simulink model "Maneuver"  (R2023b)
settings: Solver=ode4  StartTime=0.0  StopTime=30  FixedStep=dt  RelTol=1e-3
InitFcn:
  | SimulationInitialization
StopFcn:
  | SimulationEnd
values from neighbouring files (symbols this model uses):
  C = GeneticOpt.C    [SimulationCostFunction.m]
  c = Sw/b    (= 0.841696750903)    [SimulationControlConfig16P.m]    (also in SimulationControlConfig16P_LEGACY.m; SimulationControlConfigTAILLESS.m = 0.354008438819; SimulationControlConfigUTAIL.m = 0.354008438819)
  CL_Limit = CL_Max    (= 0.54)    [SimulationControlConfig16P.m]    (also in SimulationControlConfig16P_LEGACY.m; SimulationControlConfigTAILLESS.m; SimulationControlConfigUTAIL.m = 0.53)
  CL_Max_Nom = 0.465    [SimulationControlConfig16P.m]    (also in SimulationControlConfig16P_LEGACY.m; SimulationControlConfigTAILLESS.m = 0.39; SimulationControlConfigUTAIL.m)
  CL_Min = 0    [SimulationControlConfig16P.m]    (also in SimulationControlConfig16P_LEGACY.m; SimulationControlConfigTAILLESS.m; SimulationControlConfigUTAIL.m)
  dCl_per_dFlap = 0.005581818    [SimulationControlConfig16P.m]    (also in SimulationControlConfig16P_LEGACY.m = 0; SimulationControlConfigTAILLESS.m = 0; SimulationControlConfigUTAIL.m = 0)
  dt = DLLSim.dt    [SimulationTimeStep.m]    (also in SimulationTrim.m = 0.02)
  ElevatorDeflectionRate = 15    [SimulationControlConfig16P.m]    (also in SimulationControlConfig16P_LEGACY.m = 12; SimulationControlConfigTAILLESS.m = 10; SimulationControlConfigUTAIL.m = 12)
  ElevatorMax = 25    [SimulationControlConfig16P.m]    (also in SimulationControlConfig16P_LEGACY.m; SimulationControlConfigTAILLESS.m; SimulationControlConfigUTAIL.m)
  ElevatorPower = -0.002209    [SimulationControlConfig16P.m]    (also in SimulationControlConfig16P_LEGACY.m; SimulationControlConfigTAILLESS.m = -0.002956; SimulationControlConfigUTAIL.m = -0.00205983)
  ElevatorTrim = -3.5    [SimulationControlConfig16P.m]    (also in SimulationControlConfig16P_LEGACY.m; SimulationControlConfigTAILLESS.m = -6; SimulationControlConfigUTAIL.m = -8)
  Fp_Elevator = 0.55*2*pi*PitchRateLpfCutoff*dt    [SimulationControlConfig16P.m]    (also in SimulationControlConfig16P_LEGACY.m; SimulationControlConfigTAILLESS.m; SimulationControlConfigUTAIL.m)
  Fp_Pitch_2 = 0.55*2*pi*PitchBandwidth*dt    [SimulationControlConfig16P.m]    (also in SimulationControlConfig16P_LEGACY.m; SimulationControlConfigTAILLESS.m; SimulationControlConfigUTAIL.m)
  LaunchRollingElevator = -1.5    [SimulationControlConfig16P.m]    (also in SimulationControlConfig16P_LEGACY.m; SimulationControlConfigTAILLESS.m = 1; SimulationControlConfigUTAIL.m = 1)
  LiftSlope = 0.064285    [SimulationControlConfig16P.m]    (also in SimulationControlConfig16P_LEGACY.m; SimulationControlConfigTAILLESS.m = 0.058631; SimulationControlConfigUTAIL.m)
  LPFclestInit = 0    [SimulationControlPre.m]
  LPFvRate2PitchInit = 0.1    [SimulationControlPre.m]
  m = 13.1784    [InertiaEstimatorBWB.m]    (also in SimulationControlConfig16P.m = MassBWB; SimulationControlConfig16P_LEGACY.m = MassBWB; SimulationControlConfigTAILLESS.m = Weight / 2.2; SimulationControlConfigUTAIL.m = Weight / 2.2)
  nMax_User = 2.6    [SimulationControlConfig16P.m]    (also in SimulationControlConfig16P_LEGACY.m; SimulationControlConfigTAILLESS.m = 2.5; SimulationControlConfigUTAIL.m = 2.5)
  nMin_User = -1.3    [SimulationControlConfig16P.m]    (also in SimulationControlConfig16P_LEGACY.m; SimulationControlConfigTAILLESS.m = -1; SimulationControlConfigUTAIL.m = -1)
  Pitch2ElevatorIntegratorInit = -4    [SimulationControlPre.m]
  PitchDamping = -1.2608    [SimulationControlConfig16P.m]    (also in SimulationControlConfig16P_LEGACY.m; SimulationControlConfigTAILLESS.m = -0.6814; SimulationControlConfigUTAIL.m)
  PitchDampingTrust = 0.3    [SimulationControlConfig16P.m]    (also in SimulationControlConfig16P_LEGACY.m = 0.2; SimulationControlConfigTAILLESS.m = 0; SimulationControlConfigUTAIL.m = 0)
  PitchMaxAccel = 1.0    (= 1)    [SimulationControlConfig16P.m]    (also in SimulationControlConfig16P_LEGACY.m = 1.2; SimulationControlConfigTAILLESS.m; SimulationControlConfigUTAIL.m = 1.1)
  PitchRateLpfCutoff = 3    [SimulationControlConfig16P.m]    (also in SimulationControlConfig16P_LEGACY.m; SimulationControlConfigTAILLESS.m; SimulationControlConfigUTAIL.m = 5)
  PitchRateMax_User = PitchRateMax_User/180*pi    (= 0.523598775598)    [SimulationControlConfig16P.m]    (also in SimulationControlConfig16P_LEGACY.m; SimulationControlConfigTAILLESS.m; SimulationControlConfigUTAIL.m)
  PitchStiffness = -0.0041    [SimulationControlConfig16P.m]    (also in SimulationControlConfig16P_LEGACY.m; SimulationControlConfigTAILLESS.m = -0.00225; SimulationControlConfigUTAIL.m = -0.00194915)
  Q = GeneticOpt.Q    [SimulationCostFunction.m]
  R = GeneticOpt.R    [SimulationCostFunction.m]
  RateLimitPitchRateAccel = 0    [SimulationControlPre.m]
  RollingElevator = 5    [SimulationControlConfig16P.m]    (also in SimulationControlConfig16P_LEGACY.m; SimulationControlConfigTAILLESS.m = 6.5; SimulationControlConfigUTAIL.m = 7)
  RotationElevator = -6.5    [SimulationControlConfig16P.m]    (also in SimulationControlConfig16P_LEGACY.m; SimulationControlConfigTAILLESS.m = -4.25; SimulationControlConfigUTAIL.m = -5.7)
  RotationRate = (RotationElevator - LaunchRollingElevator)/RotationTime    (= -1)    [SimulationControlConfig16P.m]    (also in SimulationControlConfig16P_LEGACY.m; SimulationControlConfigTAILLESS.m = -1.5; SimulationControlConfigUTAIL.m = -1.86111111111)
  Sw = 4.663    [SimulationControlConfig16P.m]    (also in SimulationControlConfig16P_LEGACY.m; SimulationControlConfigTAILLESS.m = 0.839; SimulationControlConfigUTAIL.m = 0.839)
  taxiTrackOffset = testPlans(testIndx).rolloutTrackOffset    [SimulationControlConfig16P.m]    (also in SimulationControlConfig16P_LEGACY.m; SimulationControlConfigTAILLESS.m; SimulationControlConfigUTAIL.m)
  YInertia = 134.120    (= 134.12)    [SimulationControlConfig16P.m]    (also in SimulationControlConfig16P_LEGACY.m; SimulationControlConfigTAILLESS.m = IYY / 3417.17; SimulationControlConfigUTAIL.m = IYY / 3417.17)
undefined symbols (not defined in the file or in its folder): DiscIntNeverNeededParam, gain_resolution, K_TS, KI_Pitch, KP_Pitch, PB, pilotTime, stepTime
libraries: simulink x22, Lib_Piccolo x18, simulink_extras x1
(part 1 of 2)
settings Model: Creator=JSheng  LastModifiedBy=JCdFFigueira
settings SolverCC: AlgebraicLoopSolver=TrustRegion
settings DataIOCC: SaveFormat=Array  SignalLogging=off  DSMLogging=off  SaveTime=off  ReturnWorkspaceOutputs=off  OutputSaveName=COST
settings DebuggingCC: UnconnectedInputMsg=warning  UnconnectedOutputMsg=warning  UnconnectedLineMsg=warning  ArithmeticOperatorsInVariantConditions=warning
settings ModelReferenceCC: EnableRefExpFcnMdlSchedulingChecks=on
settings SFSimCC: CustomCodeUndefinedFunction=UseInterfaceOnly

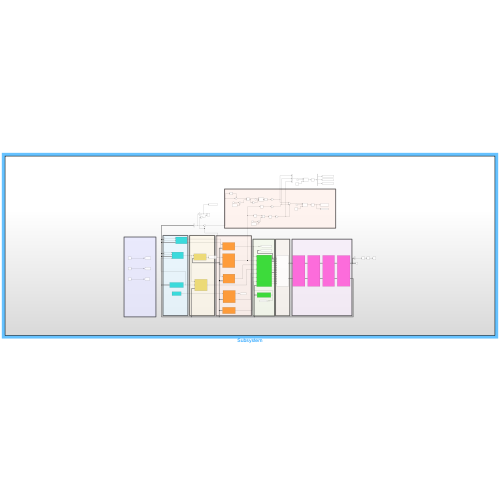
[thumbnail: Simulink's stored preview of the top-level diagram]
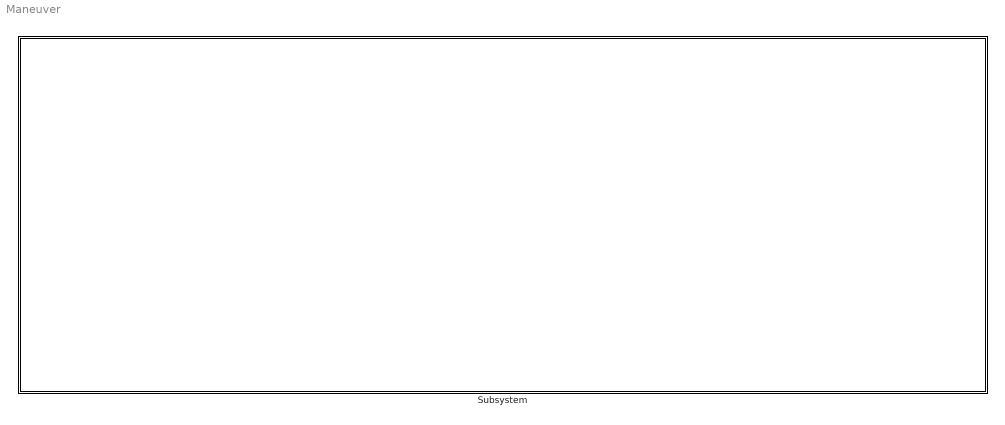
== system Maneuver ==
  Subsystem : Subsystem

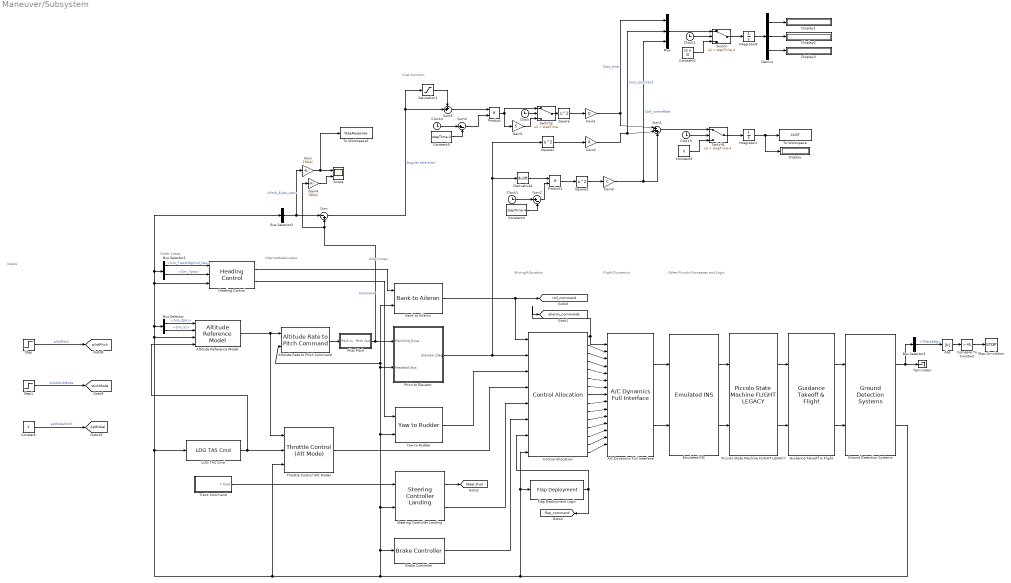
== system Maneuver/Subsystem ==
  note: Outer Loops
  note: Intermediate Loops
  note: Inner Loops
  note: Flight Dynamics
  note: Other Piccolo Processes and Logic
  note: Mixing/Allocation
  note: Inputs
  note: Cost function
  A/C Dynamics Full Interface : Lib_Piccolo/A//C Dynamics Full Interface  SystemSampleTime=-1  VariantActivationTime=update diagram  AllowFlexibleInterface=on  Latency=0  AutoFrameSizeCalculation=off
  Abs : Abs  SaturateOnIntegerOverflow=off
  Altitude Rate to Pitch Command : Lib_Piccolo/Altitude Rate to Pitch Command  SystemSampleTime=-1  VariantActivationTime=update diagram  AllowFlexibleInterface=on  Latency=0  AutoFrameSizeCalculation=off
  Altitude Reference Model : Lib_Piccolo/Altitude Reference Model  SystemSampleTime=-1  VariantActivationTime=update diagram  AllowFlexibleInterface=on  Latency=0  AutoFrameSizeCalculation=off
  Bank to Aileron : Lib_Piccolo/Bank to Aileron  SystemSampleTime=-1  VariantActivationTime=update diagram  AllowFlexibleInterface=on  Latency=0  AutoFrameSizeCalculation=off
  Brake Controller : Lib_Piccolo/Brake Controller  SystemSampleTime=-1  VariantActivationTime=update diagram  AllowFlexibleInterface=on  Latency=0  AutoFrameSizeCalculation=off
  Bus Selector : BusSelector  OutputSignals=Sim_Zpos,Sim_Vz
  Bus Selector1 : BusSelector  OutputSignals=Sim_TrackHdgCmd_Deg,Sim_Ypos
  Bus Selector2 : BusSelector  OutputSignals=Pitch_Euler_rad
  Bus Selector3 : BusSelector  OutputSignals=ThetaDeg
  Clock{,1..4} (5 alike) : Clock
  Compare To Constant : simulink/Logic and Bit Operations/Compare To Constant  relop=>  const=45  OutDataTypeStr=boolean
  Constant : Constant
  Constant2 : Constant  Value=[0 0 0]
  Constant3 : Constant  Value=0
  Constant4 : Constant  Value=stepTime-4
  Constant5 : Constant  Value=stepTime-4
  Control Allocation : Lib_Piccolo/Control Allocation  SystemSampleTime=-1  VariantActivationTime=update diagram  AllowFlexibleInterface=on  Latency=0  AutoFrameSizeCalculation=off
  Demux : Demux  Outputs=3
  Derivative1 : Derivative
  Display{,1..3} (4 alike) : Display
  Emulated INS : Lib_Piccolo/Emulated INS  SystemSampleTime=-1  VariantActivationTime=update diagram  AllowFlexibleInterface=on  Latency=0  AutoFrameSizeCalculation=off
  Flap Deployment Logic : Lib_Piccolo/Flap Deployment  SystemSampleTime=-1  VariantActivationTime=update diagram  AllowFlexibleInterface=on  Latency=0  AutoFrameSizeCalculation=off
  Gain : Gain  Gain=180/pi
  Gain1 : Gain  Gain=Q
  Gain2 : Gain  Gain=R
  Gain3 : Gain  Gain=C
  Gain4 : Gain  Gain=180/pi
  Gain5 : Gain  Gain=5
  Ground Detection Systems : Lib_Piccolo/Ground Detection Systems  SystemSampleTime=-1  VariantActivationTime=update diagram  AllowFlexibleInterface=on  Latency=0  AutoFrameSizeCalculation=off
  Guidance Takeoff & Flight : Lib_Piccolo/Guidance Takeoff & Flight  SystemSampleTime=-1  VariantActivationTime=update diagram  AllowFlexibleInterface=on  Latency=0  AutoFrameSizeCalculation=off
  Heading Control : Lib_Piccolo/Heading Control  SystemSampleTime=-1  VariantActivationTime=update diagram  AllowFlexibleInterface=on  Latency=0  AutoFrameSizeCalculation=off
  Integrator1 : Integrator
  Integrator6 : Integrator
  LDG TAS Cmd : Lib_Piccolo/LDG TAS Cmd  SystemSampleTime=-1  VariantActivationTime=update diagram  AllowFlexibleInterface=on  Latency=0  AutoFrameSizeCalculation=off
  Mux : Mux  Inputs=3
  Piccolo State Machine FLIGHT LEGACY : Lib_Piccolo/Piccolo State Machine FLIGHT LEGACY  SystemSampleTime=-1  VariantActivationTime=update diagram  AllowFlexibleInterface=on  Latency=0  AutoFrameSizeCalculation=off
  Pilot Pitch : Subsystem
  Pitch to Elevator : Subsystem  AncestorBlock=Lib_Piccolo/Pitch to Elevator
  Product : Product
  Product1 : Product
  Saturation1 : Saturate  UpperLimit=0  LowerLimit=-inf
  Scope : Scope  NumInputPorts=2
  Square : Math  Operator=square
  Square1 : Math  Operator=square
  Square2 : Math  Operator=square
  Steering Controller Landing : Lib_Piccolo/Steering Controller Landing  SystemSampleTime=-1  VariantActivationTime=update diagram  AllowFlexibleInterface=on  Latency=0  AutoFrameSizeCalculation=off
  Step : Step  Time=stepTime  Before=4.97  After=6.97  SampleTime=dt
  Step1 : Step  Time=pilotTime  SampleTime=dt
  Stop Simulation : Stop
  Sum : Sum  Inputs=|-+
  Sum1 : Sum  Inputs=|+++
  Sum2 : Sum  Inputs=|+-
  Sum3 : Sum  Inputs=++|
  Sum4 : Sum  Inputs=|+-
  Switch : Switch  Criteria=u2 > Threshold  Threshold=stepTime-4  SaturateOnIntegerOverflow=off  InputSameDT=off
  Switch1 : Switch  Criteria=u2 > Threshold  Threshold=stepTime-4  SaturateOnIntegerOverflow=off  InputSameDT=off
  Switch2 : Switch  Criteria=u2 > Threshold  Threshold=stepTime  SaturateOnIntegerOverflow=off  InputSameDT=off
  Terminator : Terminator
  Throttle Control (Alt Mode) : Lib_Piccolo/Throttle Control (Alt Mode)  SystemSampleTime=-1  VariantActivationTime=update diagram  AllowFlexibleInterface=on  Latency=0  AutoFrameSizeCalculation=off
  To Workspace : ToWorkspace  VariableName=COST  SaveFormat=Timeseries  SampleTime=-1
  To Workspace1 : ToWorkspace  VariableName=StepResponse  SaveFormat=Timeseries  SampleTime=-1
  Track Command : Subsystem
  Yaw to Rudder : Lib_Piccolo/Yaw to Rudder  SystemSampleTime=-1  VariantActivationTime=update diagram  AllowFlexibleInterface=on  Latency=0  AutoFrameSizeCalculation=off
  tag scope: ApGlobal=global, Steer_Rud=global, aileron_commands=global, flap_command=global, pilotPitch=global, roll_command=global, stickMode=global
  wires:
  Bus Selector/2 -> Altitude Reference Model/2  "<Sim_Vz>"
  Control Allocation/6 -> A/C Dynamics Full Interface/6
  Control Allocation/9 -> A/C Dynamics Full Interface/9
  Control Allocation/7 -> A/C Dynamics Full Interface/7
  Control Allocation/8 -> A/C Dynamics Full Interface/8
  Ground Detection Systems/2 -> LDG TAS Cmd/1, Bus Selector/1, Heading Control/3, Bus Selector2/1, Bus Selector1/1, Altitude Reference Model/3, Throttle Control (Alt Mode)/3, Bank to Aileron/2, Altitude Rate to Pitch Command/2, Pitch to Elevator/2(Feedback Bus), Yaw to Rudder/2, Steering Controller Landing/2, Brake Controller/1, Flap Deployment Logic/1, Control Allocation/8
  Control Allocation/3 -> A/C Dynamics Full Interface/3
  Control Allocation/11 -> A/C Dynamics Full Interface/11
  A/C Dynamics Full Interface/2 -> Emulated INS/2
  Bus Selector/1 -> Altitude Reference Model/1  "<Sim_Zpos>"
  Control Allocation/4 -> A/C Dynamics Full Interface/4
  Flap Deployment Logic/1 -> [flap_command], Control Allocation/7
  Control Allocation/13 -> A/C Dynamics Full Interface/13
  Heading Control/2 -> Yaw to Rudder/1
  Control Allocation/5 -> A/C Dynamics Full Interface/5
  A/C Dynamics Full Interface/1 -> Emulated INS/1
  Control Allocation/14 -> A/C Dynamics Full Interface/14
  Piccolo State Machine FLIGHT LEGACY/2 -> Guidance Takeoff & Flight/2
  Bus Selector1/1 -> Heading Control/1  "<Sim_TrackHdgCmd_Deg>"
  Steering Controller Landing/1 -> [Steer_Rud]
  LDG TAS Cmd/1 -> Throttle Control (Alt Mode)/2, Altitude Reference Model/4
  Brake Controller/1 -> Control Allocation/6
  Altitude Rate to Pitch Command/1 -> Pilot Pitch/1(Pitch In)
  Track Command/1(Y Cmd) -> Steering Controller Landing/1
  Emulated INS/1 -> Piccolo State Machine FLIGHT LEGACY/1
  Control Allocation/2 -> A/C Dynamics Full Interface/2
  Guidance Takeoff & Flight/1 -> Ground Detection Systems/1
  Emulated INS/2 -> Piccolo State Machine FLIGHT LEGACY/2
  Piccolo State Machine FLIGHT LEGACY/1 -> Guidance Takeoff & Flight/1
  Control Allocation/12 -> A/C Dynamics Full Interface/12
  Control Allocation/10 -> A/C Dynamics Full Interface/10
  Guidance Takeoff & Flight/2 -> Ground Detection Systems/2
  Bus Selector1/2 -> Heading Control/2  "<Sim_Ypos>"
  Control Allocation/15 -> A/C Dynamics Full Interface/15
  Steering Controller Landing/2 -> Control Allocation/5
  Ground Detection Systems/1 -> Bus Selector3/1, Terminator/1
  Control Allocation/1 -> [aileron_commands], A/C Dynamics Full Interface/1
  Bank to Aileron/1 -> Control Allocation/1, [roll_command]
  Pitch to Elevator/1(Elevator_Deg) -> Square1/1, Derivative1/1, Control Allocation/2
  Yaw to Rudder/1 -> Control Allocation/3
  Throttle Control (Alt Mode)/1 -> Control Allocation/4
  Heading Control/1 -> Bank to Aileron/1
  Altitude Reference Model/1 -> Altitude Rate to Pitch Command/1, Throttle Control (Alt Mode)/1
  Constant/1 -> [ApGlobal]  "apGlobalCmd"
  Step/1 -> [pilotPitch]  "pilotPitch"
  Step1/1 -> [stickMode]  "pilotStickMode"
  Pilot Pitch/1(Pitch Out) -> Pitch to Elevator/1(PitchCmd_Euler), Gain4/1, Sum/2  "Command"
  Saturation1/1 -> Sum3/1
  Square2/1 -> Gain3/1
  Square1/1 -> Gain2/1
  Gain1/1 -> Mux/1, Sum1/1  "Cost_error"
  Sum/1 -> Sum3/2, Saturation1/1  "Angular rate error"
  Product1/1 -> Square2/1
  Gain3/1 -> Mux/3, Sum1/3  "Cost_commRate"
  Square/1 -> Gain1/1
  Clock1/1 -> Sum2/1
  Product/1 -> Gain5/1, Switch2/1
  Derivative1/1 -> Product1/1
  Gain2/1 -> Mux/2, Sum1/2  "Cost_command"
  Bus Selector2/1 -> Gain/1, Sum/1  "<Pitch_Euler_rad>"
  Clock2/1 -> Switch/2
  Constant2/1 -> Switch/3
  Mux/1 -> Switch/1
  Integrator6/1 -> Demux/1
  Demux/1 -> Display1/1
  Demux/2 -> Display2/1
  Demux/3 -> Display3/1
  Constant3/1 -> Switch1/3
  Clock3/1 -> Switch1/2
  Sum1/1 -> Switch1/1
  Integrator1/1 -> Display/1, To Workspace/1
  Sum2/1 -> Product1/2
  Constant4/1 -> Sum2/2
  Clock4/1 -> Sum4/1
  Sum4/1 -> Product/2
  Constant5/1 -> Sum4/2
  Gain/1 -> To Workspace1/1, Scope/1
  Gain4/1 -> Scope/2
  Bus Selector3/1 -> Abs/1  "<ThetaDeg>"
  Compare To Constant/1 -> Stop Simulation/1
  Abs/1 -> Compare To Constant/1
  Sum3/1 -> Product/1
  Switch/1 -> Integrator6/1
  Switch1/1 -> Integrator1/1
  Clock/1 -> Switch2/2
  Switch2/1 -> Square/1
  Gain5/1 -> Switch2/3

== system Maneuver/Subsystem/Pilot Pitch ==
  Pitch In : Inport
  Degrees to Radians1 : simulink_extras/Transformations/Degrees to Radians
  Switch3 : Switch  Criteria=u2 > Threshold  SaturateOnIntegerOverflow=off  InputSameDT=off
  Pitch Out : Outport  VectorParamsAs1DForOutWhenUnconnected=off
  wires:
  [stickMode] -> Switch3/2
  Degrees to Radians1/1 -> Switch3/1
  Pitch In/1 -> Switch3/3
  [pilotPitch] -> Degrees to Radians1/1
  Switch3/1 -> Pitch Out/1

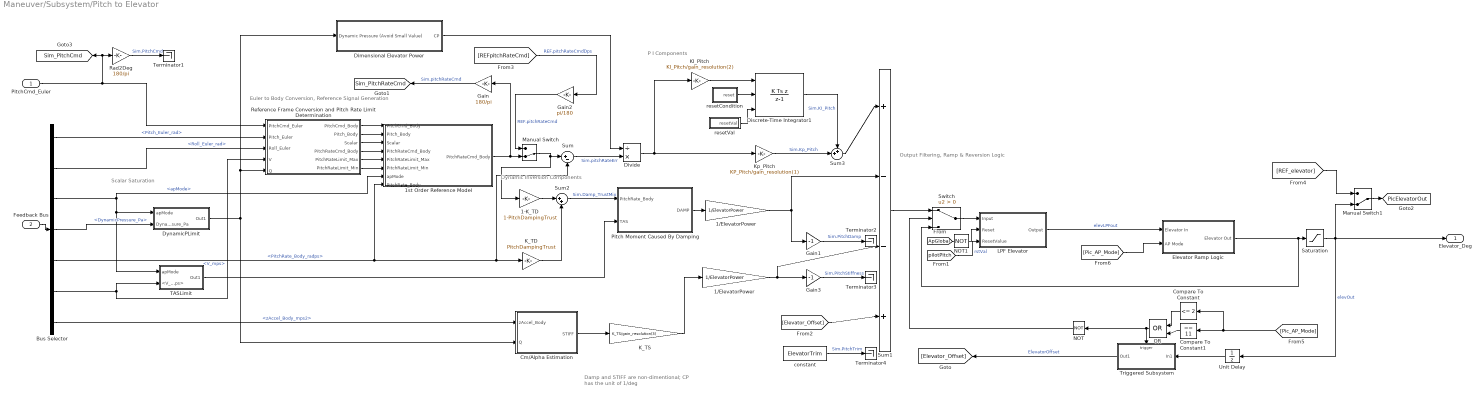
== system Maneuver/Subsystem/Pitch to Elevator ==
  note: Damp and STIFF are non-dimentional;
      | CP has the unit of 1/deg
  note: P I Components
  note: Dynamic Inversion Components
  note: Output Filtering, Ramp & Reversion Logic
  note: Scalar Saturation
  note: Euler to Body Conversion, Reference Signal Generation
  PitchCmd_Euler : Inport
  Feedback Bus : Inport  Port=2
  1-K_TD : Gain  Gain=1-PitchDampingTrust
  1/ElevatorPower : Gain  Gain=1/ElevatorPower
  "1/ElevatorPower  " : Gain  Gain=1/ElevatorPower
  1st Order Reference Model : Subsystem
  Bus Selector : BusSelector  OutputSignals=Pitch_Euler_rad,Roll_Euler_rad,apMode,DynamicPressure_Pa,PitchRate_Body_radps,V_mps,zAccel_Body_mps2
  Cm/Alpha Estimation : Subsystem
  Compare To Constant : simulink/Logic and Bit Operations/Compare To Constant  relop=<=  const=2  OutDataTypeStr=boolean
  Compare To Constant1 : simulink/Logic and Bit Operations/Compare To Constant  relop===  const=11  OutDataTypeStr=uint8
  Dimensional Elevator Power : Subsystem
  Discrete-Time Integrator1 : DiscreteIntegrator  IntegratorMethod=Integration: Backward Euler  ExternalReset=level  InitialConditionSource=external  SampleTime=-1  LimitOutput=on  UpperSaturationLimit=ElevatorMax  LowerSaturationLimit=-ElevatorMax  ICPrevOutput=DiscIntNeverNeededParam  ICPrevScaledInput=DiscIntNeverNeededParam
  Divide : Product  Inputs=/*
  DynamicPLimit : Subsystem
  Elevator Ramp Logic : Subsystem
  Gain : Gain  Gain=180/pi
  Gain1 : Gain  Gain=-1
  Gain2 : Gain  Gain=pi/180
  Gain3 : Gain  Gain=-1
  KI_Pitch : Gain  Gain=KI_Pitch/gain_resolution(2)
  K_TD : Gain  Gain=PitchDampingTrust
  K_TS : Gain  Gain=K_TS/gain_resolution(3)
  Kp_Pitch : Gain  Gain=KP_Pitch/gain_resolution(1)
  LPF Elevator : Subsystem
  Manual Switch : ManualSwitch  CurrentSetting=0
  Manual Switch1 : ManualSwitch  CurrentSetting=0
  NOT : Logic  Operator=NOT  IconShape=distinctive  AllPortsSameDT=off  OutDataTypeStr=boolean
  NOT1 : Logic  Operator=NOT  IconShape=distinctive  AllPortsSameDT=off  OutDataTypeStr=boolean
  OR : Logic  Operator=OR  IconShape=distinctive  AllPortsSameDT=off  OutDataTypeStr=boolean
  Pitch Moment Caused By Damping : Subsystem
  Rad2Deg : Gain  Gain=180/pi
  Reference Frame Conversion and Pitch Rate Limit Determination : Subsystem
  Saturation : Saturate  UpperLimit=ElevatorMax  LowerLimit=-ElevatorMax
  Sum : Sum  Inputs=|+-
  Sum1 : Sum  Inputs=|+--+
  Sum2 : Sum  Inputs=|++
  Sum3 : Sum  Inputs=++|
  Switch : Switch  Criteria=u2 > Threshold  SaturateOnIntegerOverflow=off  InputSameDT=off
  TASLimit : Subsystem
  Terminator{1..4} (4 alike) : Terminator
  Triggered Subsystem : Subsystem  TreatAsAtomicUnit=on
  Unit Delay : UnitDelay  SampleTime=-1  HasFrameUpgradeWarning=on
  constant : Constant  Value=ElevatorTrim  VectorParams1D=off
  resetCondition : Subsystem
  resetVal : Subsystem
  Elevator_Deg : Outport  VectorParamsAs1DForOutWhenUnconnected=off
  tag scope: PicElevatorOut=global, Sim_PitchCmd=global, Sim_PitchRateCmd=global
  wires:
  K_TS/1 -> "1/ElevatorPower  "/1
  [Pic_AP_Mode] -> Elevator Ramp Logic/2(AP Mode)
  LPF Elevator/1(Output) -> Elevator Ramp Logic/1(Elevator In)  "elevLPFout"
  Elevator Ramp Logic/1(Elevator Out) -> Saturation/1, Switch/3
  [REF_elevator] -> Manual Switch1/1
  Manual Switch1/1 -> [PicElevatorOut]
  resetVal/1(resetVal) -> Discrete-Time Integrator1/3
  [pilotPitch] -> LPF Elevator/3(ResetValue)  "rstVal"
  NOT1/1 -> LPF Elevator/2(Reset)
  [ApGlobal] -> NOT1/1
  Reference Frame Conversion and Pitch Rate Limit Determination/1(PitchCmd_Body) -> 1st Order Reference Model/1(PitchCmd_Body)
  Sum/1 -> Divide/2  "Sim.pitchRateErr"
  1st Order Reference Model/1(PitchRateCmd_Body) -> Manual Switch/2, Gain/1
  1-K_TD/1 -> Sum2/1
  K_TD/1 -> Sum2/2
  Cm/Alpha Estimation/1(STIFF) -> K_TS/1
  Reference Frame Conversion and Pitch Rate Limit Determination/2("Pitch_Body ") -> 1st Order Reference Model/2("Pitch_Body ")
  Dimensional Elevator Power/1(CP) -> Divide/1
  PitchCmd_Euler/1 -> Reference Frame Conversion and Pitch Rate Limit Determination/1(PitchCmd_Euler), Rad2Deg/1, [Sim_PitchCmd]
  Reference Frame Conversion and Pitch Rate Limit Determination/4(PitchRateCmd_Body) -> 1st Order Reference Model/4("PitchRateCmd_Body ")
  Reference Frame Conversion and Pitch Rate Limit Determination/6("PitchRateLimit_Min ") -> 1st Order Reference Model/6(" PitchRateLimit_Min ")
  Feedback Bus/1 -> Bus Selector/1
  Bus Selector/1 -> Reference Frame Conversion and Pitch Rate Limit Determination/2(Pitch_Euler)  "<Pitch_Euler_rad>"
  Bus Selector/2 -> Reference Frame Conversion and Pitch Rate Limit Determination/3(Roll_Euler)  "<Roll_Euler_rad>"
  Bus Selector/5 -> K_TD/1, Sum/2, 1st Order Reference Model/8(PitchRate_Body)  "<PitchRate_Body_radps>"
  Bus Selector/7 -> Cm/Alpha Estimation/1(zAccel_Body)  "<zAccel_Body_mps2>"
  Sum1/1 -> Switch/1
  "1/ElevatorPower  "/1 -> Gain3/1, Sum1/3
  Gain3/1 -> Terminator3/1  "Sim.PitchStiffness"
  Gain1/1 -> Terminator2/1  "Sim.PitchDamp"
  Gain/1 -> [Sim_PitchRateCmd]  "Sim.pitchRateCmd"
  Bus Selector/3 -> DynamicPLimit/1(apMode), TASLimit/1(apMode), 1st Order Reference Model/7(apMode)  "<apMode>"
  KI_Pitch/1 -> Discrete-Time Integrator1/1
  Divide/1 -> Kp_Pitch/1, KI_Pitch/1
  Sum3/1 -> Sum1/1
  Kp_Pitch/1 -> Sum3/2  "Sim.Kp_Pitch"
  Discrete-Time Integrator1/1 -> Sum3/1  "Sim.KI_Pitch"
  constant/1 -> Terminator4/1  "Sim.PitchTrim"
  Pitch Moment Caused By Damping/1(DAMP) -> 1/ElevatorPower/1
  [REFpitchRateCmd] -> Gain2/1  "REF.pitchRateCmdDps"
  Manual Switch/1 -> 1-K_TD/1, Sum/1
  Gain2/1 -> Manual Switch/1  "REF.pitchRateCmd"
  1/ElevatorPower/1 -> Gain1/1, Sum1/2
  Sum2/1 -> Pitch Moment Caused By Damping/1(PitchRate_Body)  "Sim.Damp_TrustMix"
  Reference Frame Conversion and Pitch Rate Limit Determination/5("PitchRateLimit_Max ") -> 1st Order Reference Model/5("PitchRateLimit_Max ")
  Reference Frame Conversion and Pitch Rate Limit Determination/3("Scalar ") -> 1st Order Reference Model/3("Scalar ")
  [Elevator_Offset] -> Sum1/4
  Saturation/1 -> Manual Switch1/2, Elevator_Deg/1, Unit Delay/1  "elevOut"
  Unit Delay/1 -> Triggered Subsystem/1(In1)
  Triggered Subsystem/1(Out1) -> [Elevator_Offset]  "ElevatorOffset"
  Switch/1 -> LPF Elevator/1(Input)
  NOT/1 -> Switch/2
  [Pic_AP_Mode] -> Compare To Constant/1, Compare To Constant1/1
  DynamicPLimit/1(Out1) -> Dimensional Elevator Power/1(Dynamic Pressure (Avoid Small Value)), Reference Frame Conversion and Pitch Rate Limit Determination/5(Q), Cm/Alpha Estimation/2(Q)
  Bus Selector/4 -> DynamicPLimit/2(DynamicPressure_Pa)  "<DynamicPressure_Pa>"
  TASLimit/1(Out1) -> Pitch Moment Caused By Damping/2(TAS)
  Bus Selector/6 -> TASLimit/2(<V_mps>), Reference Frame Conversion and Pitch Rate Limit Determination/4(V)  "<V_mps>"
  resetCondition/1(reset) -> Discrete-Time Integrator1/2
  Rad2Deg/1 -> Terminator1/1  "Sim.PitchCmd"
  Compare To Constant/1 -> OR/1
  OR/1 -> NOT/1, Triggered Subsystem/Trigger
  Compare To Constant1/1 -> OR/2

== system Maneuver/Subsystem/Track Command ==
  In-Flight Cmd : Constant  Value=taxiTrackOffset
  Switch : Switch  Threshold=11  SaturateOnIntegerOverflow=off  InputSameDT=off
  Taxi Cmd : Constant  Value=taxiTrackOffset
  Y Cmd : Outport  VectorParamsAs1DForOutWhenUnconnected=off
  wires:
  [Pic_AP_Mode] -> Switch/2
  Switch/1 -> Y Cmd/1
  Taxi Cmd/1 -> Switch/1
  In-Flight Cmd/1 -> Switch/3

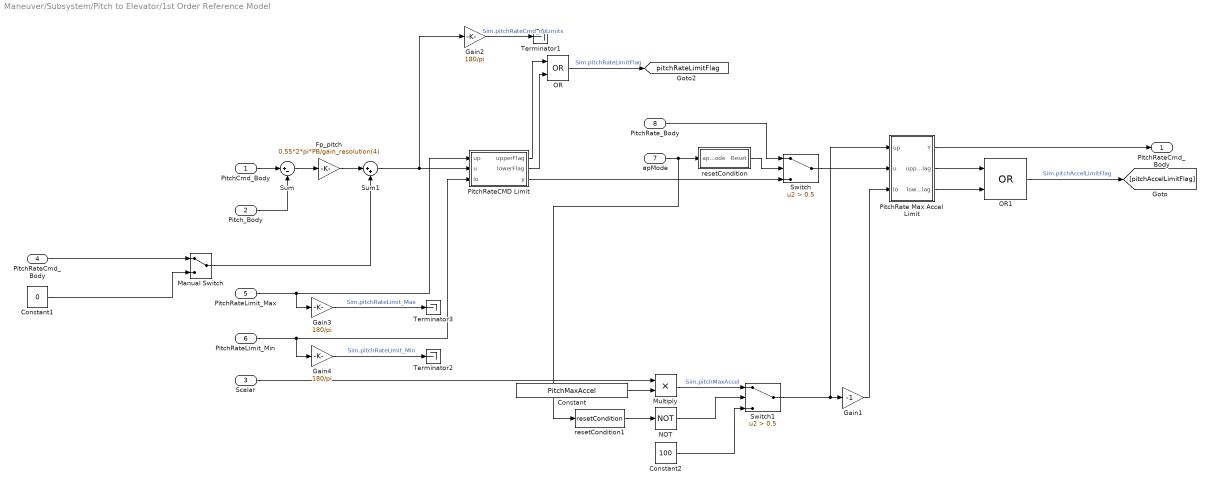
== system Maneuver/Subsystem/Pitch to Elevator/1st Order Reference Model ==
  PitchCmd_Body : Inport
  "Pitch_Body " : Inport  Port=2
  "Scalar " : Inport  Port=3
  "PitchRateCmd_Body " : Inport  Port=4
  "PitchRateLimit_Max " : Inport  Port=5
  " PitchRateLimit_Min " : Inport  Port=6
  apMode : Inport  Port=7
  PitchRate_Body : Inport  Port=8
  Constant : Constant  Value=PitchMaxAccel
  Constant1 : Constant  Value=0
  Constant2 : Constant  Value=100
  Fp_pitch : Gain  Gain=0.55*2*pi*PB/gain_resolution(4)
  Gain1 : Gain  Gain=-1
  Gain2 : Gain  Gain=180/pi
  Gain3 : Gain  Gain=180/pi
  Gain4 : Gain  Gain=180/pi
  Manual Switch : ManualSwitch
  Multiply : Product
  NOT : Logic  Operator=NOT  IconShape=distinctive  AllPortsSameDT=off  OutDataTypeStr=boolean
  OR : Logic  Operator=OR  IconShape=distinctive  AllPortsSameDT=off  OutDataTypeStr=boolean
  OR1 : Logic  Operator=OR  IconShape=distinctive  AllPortsSameDT=off  OutDataTypeStr=boolean
  PitchRate Max Accel Limit : Subsystem
  PitchRateCMD Limit : Subsystem
  Sum : Sum  Inputs=|+-
  Sum1 : Sum  Inputs=|++
  Switch : Switch  Criteria=u2 > Threshold  Threshold=0.5  SaturateOnIntegerOverflow=off  InputSameDT=off
  Switch1 : Switch  Criteria=u2 > Threshold  Threshold=0.5  SaturateOnIntegerOverflow=off  InputSameDT=off
  Terminator1 : Terminator
  Terminator2 : Terminator
  Terminator3 : Terminator
  resetCondition : Subsystem
  resetCondition1 : Lib_Piccolo/Pitch to Elevator/1st Order Reference Model/resetCondition  SystemSampleTime=-1  VariantActivationTime=update diagram  AllowFlexibleInterface=on  Latency=0  AutoFrameSizeCalculation=off
  PitchRateCmd_Body : Outport  VectorParamsAs1DForOutWhenUnconnected=off
  tag scope: pitchRateLimitFlag=global
  wires:
  OR1/1 -> [pitchAccelLimitFlag]  "Sim.pitchAccelLimitFlag"
  PitchRate Max Accel Limit/3(lowerFlag) -> OR1/2
  PitchRate Max Accel Limit/2(upperFlag) -> OR1/1
  Constant2/1 -> Switch1/3
  NOT/1 -> Switch1/2
  Multiply/1 -> Switch1/1  "Sim.pitchMaxAccel"
  PitchCmd_Body/1 -> Sum/1
  "Pitch_Body "/1 -> Sum/2
  Sum/1 -> Fp_pitch/1
  Fp_pitch/1 -> Sum1/1
  "Scalar "/1 -> Multiply/1
  Switch1/1 -> PitchRate Max Accel Limit/1(up), Gain1/1
  Constant/1 -> Multiply/2
  Gain1/1 -> PitchRate Max Accel Limit/3(lo)
  "PitchRateLimit_Max "/1 -> PitchRateCMD Limit/1(up), Gain3/1
  " PitchRateLimit_Min "/1 -> PitchRateCMD Limit/3(lo), Gain4/1
  Manual Switch/1 -> Sum1/2
  Constant1/1 -> Manual Switch/2
  "PitchRateCmd_Body "/1 -> Manual Switch/1
  Sum1/1 -> PitchRateCMD Limit/2(u), Gain2/1
  Gain2/1 -> Terminator1/1  "Sim.pitchRateCmd_noLimits"
  Gain4/1 -> Terminator2/1  "Sim.pitchRateLimit_Min"
  Gain3/1 -> Terminator3/1  "Sim.pitchRateLimit_Max"
  PitchRateCMD Limit/3(y) -> Switch/3
  PitchRate_Body/1 -> Switch/1
  PitchRateCMD Limit/1(upperFlag) -> OR/1
  PitchRateCMD Limit/2(lowerFlag) -> OR/2
  OR/1 -> [pitchRateLimitFlag]  "Sim.pitchRateLimitFlag"
  Switch/1 -> PitchRate Max Accel Limit/2(u)
  PitchRate Max Accel Limit/1(Y) -> PitchRateCmd_Body/1
  apMode/1 -> resetCondition/1(apMode), resetCondition1/1
  resetCondition/1(Reset) -> Switch/2
  resetCondition1/1 -> NOT/1

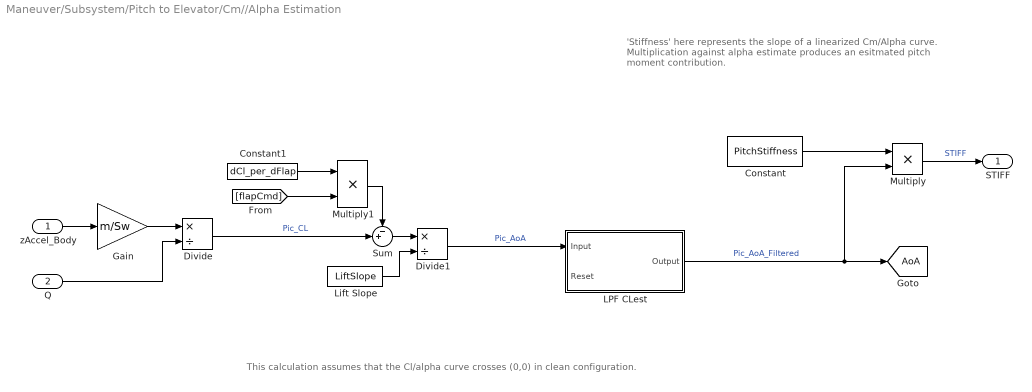
== system Maneuver/Subsystem/Pitch to Elevator/Cm//Alpha Estimation ==
  note: This calculation assumes that the Cl/alpha curve crosses (0,0) in clean configuration.
  note: 'Stiffness' here represents the slope of a linearized Cm/Alpha curve. Multiplication against alpha estimate produces an esitmated pitch moment contribution.
  zAccel_Body : Inport
  Q : Inport  Port=2
  Constant : Constant  Value=PitchStiffness
  Constant1 : Constant  Value=dCl_per_dFlap
  Divide : Product  Inputs=*/
  Divide1 : Product  Inputs=*/
  Gain : Gain  Gain=m/Sw
  LPF CLest : Subsystem
  Lift Slope : Constant  Value=LiftSlope
  Multiply : Product
  Multiply1 : Product
  Sum : Sum  Inputs=-+|
  STIFF : Outport  VectorParamsAs1DForOutWhenUnconnected=off
  tag scope: AoA=global
  wires:
  Constant/1 -> Multiply/1
  Multiply/1 -> STIFF/1  "STIFF"
  Gain/1 -> Divide/1
  Q/1 -> Divide/2
  Lift Slope/1 -> Divide1/2
  Divide/1 -> Sum/2  "Pic_CL"
  zAccel_Body/1 -> Gain/1
  LPF CLest/1(Output) -> Multiply/2, [AoA]  "Pic_AoA_Filtered"
  [flapCmd] -> Multiply1/2
  Constant1/1 -> Multiply1/1
  Multiply1/1 -> Sum/1
  Sum/1 -> Divide1/1
  Divide1/1 -> LPF CLest/1(Input)  "Pic_AoA"

== system Maneuver/Subsystem/Pitch to Elevator/Dimensional Elevator Power ==
  Dynamic Pressure (Avoid Small Value) : Inport
  Average Wing Chord : Constant  Value=c
  Multiply : Product  Inputs=****/
  Unit: Per Deg : Constant  Value=ElevatorPower
  Wing Area : Constant  Value=Sw
  YInertia : Constant  Value=YInertia
  CP : Outport  VectorParamsAs1DForOutWhenUnconnected=off
  wires:
  Dynamic Pressure (Avoid Small Value)/1 -> Multiply/1
  Wing Area/1 -> Multiply/2
  Average Wing Chord/1 -> Multiply/3
  YInertia/1 -> Multiply/5
  Multiply/1 -> CP/1
  Unit: Per Deg/1 -> Multiply/4

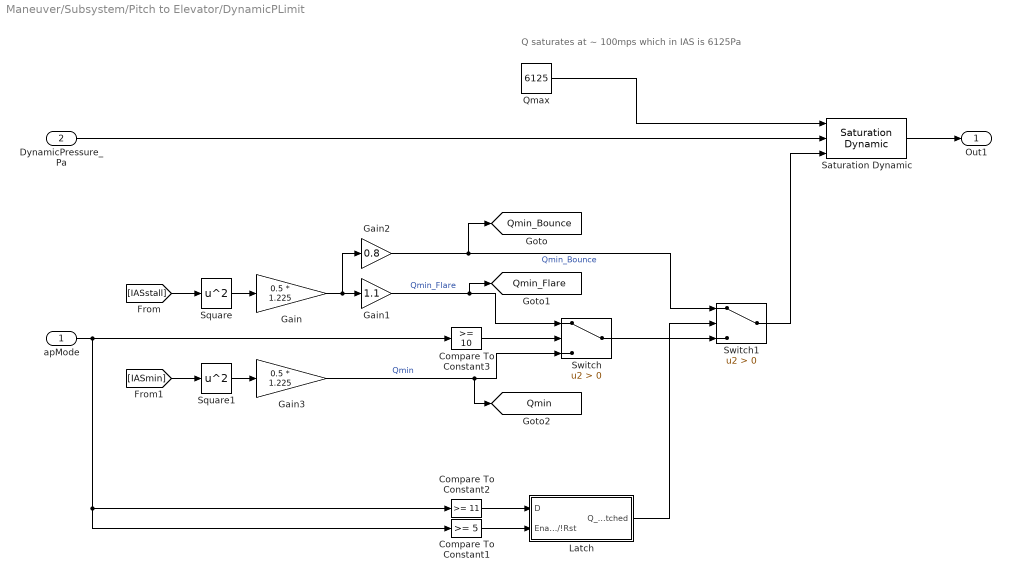
== system Maneuver/Subsystem/Pitch to Elevator/DynamicPLimit ==
  note: Q saturates at ~ 100mps which in IAS is 6125Pa
  apMode : Inport
  DynamicPressure_Pa : Inport  Port=2
  Compare To Constant1 : simulink/Logic and Bit Operations/Compare To Constant  relop=>=  const=5  OutDataTypeStr=uint8
  Compare To Constant2 : simulink/Logic and Bit Operations/Compare To Constant  relop=>=  const=11  OutDataTypeStr=uint8
  Compare To Constant3 : simulink/Logic and Bit Operations/Compare To Constant  relop=>=  const=10  OutDataTypeStr=uint8
  Gain : Gain  Gain=0.5 * 1.225
  Gain1 : Gain  Gain=1.1
  Gain2 : Gain  Gain=0.8
  Gain3 : Gain  Gain=0.5 * 1.225
  Latch : Subsystem
  Qmax : Constant  Value=6125
  Saturation Dynamic : simulink/Discontinuities/Saturation Dynamic  OutMin=[]  OutMax=[]  OutDataTypeStr=Inherit: Same as second input  OutDataType=fixdt(1, 16)  OutScaling=2^-10  DoSatur=off
  Square : Math  Operator=square  SignedPower=on
  Square1 : Math  Operator=square  SignedPower=on
  Switch : Switch  Criteria=u2 > Threshold  SaturateOnIntegerOverflow=off  InputSameDT=off
  Switch1 : Switch  Criteria=u2 > Threshold  SaturateOnIntegerOverflow=off  InputSameDT=off
  Out1 : Outport  VectorParamsAs1DForOutWhenUnconnected=off
  tag scope: Qmin=global, Qmin_Bounce=global, Qmin_Flare=global
  wires:
  DynamicPressure_Pa/1 -> Saturation Dynamic/2
  Saturation Dynamic/1 -> Out1/1
  apMode/1 -> Compare To Constant3/1, Compare To Constant2/1, Compare To Constant1/1
  Compare To Constant3/1 -> Switch/2
  Gain3/1 -> [Qmin], Switch/3  "Qmin"
  Gain1/1 -> [Qmin_Flare], Switch/1  "Qmin_Flare"
  Qmax/1 -> Saturation Dynamic/1
  Compare To Constant1/1 -> Latch/2(Enable/!Rst)
  Compare To Constant2/1 -> Latch/1(D)
  Switch/1 -> Switch1/3
  Gain2/1 -> [Qmin_Bounce], Switch1/1  "Qmin_Bounce"
  Switch1/1 -> Saturation Dynamic/3
  Latch/1(Q_Latched) -> Switch1/2
  Square/1 -> Gain/1
  [IASstall] -> Square/1
  Gain/1 -> Gain2/1, Gain1/1
  [IASmin] -> Square1/1
  Square1/1 -> Gain3/1

== system Maneuver/Subsystem/Pitch to Elevator/Elevator Ramp Logic ==
  Elevator In : Inport
  AP Mode : Inport  Port=2
  Elevator DeRotation Ramp : Subsystem
  Elevator Rotation Ramp : Subsystem
  Elevator Out : Outport  VectorParamsAs1DForOutWhenUnconnected=off
  wires:
  AP Mode/1 -> Elevator Rotation Ramp/2(apMode In), Elevator DeRotation Ramp/2(apMode In)
  Elevator In/1 -> Elevator DeRotation Ramp/1(Elevator In)
  Elevator DeRotation Ramp/1(Elevator Out) -> Elevator Rotation Ramp/1(Elevator In)
  Elevator Rotation Ramp/1(Elevator Out) -> Elevator Out/1

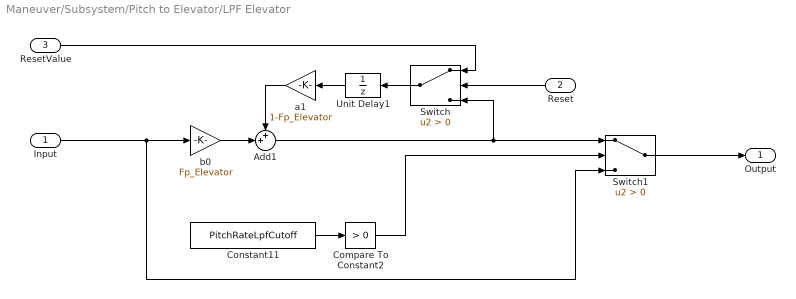
== system Maneuver/Subsystem/Pitch to Elevator/LPF Elevator ==
  Input : Inport
  Reset : Inport  Port=2
  ResetValue : Inport  Port=3
  Add1 : Sum  Inputs=++|
  Compare To Constant2 : simulink/Logic and Bit Operations/Compare To Constant  relop=>  const=0  OutDataTypeStr=uint8
  Constant11 : Constant  Value=PitchRateLpfCutoff
  Switch : Switch  Criteria=u2 > Threshold  SaturateOnIntegerOverflow=off  InputSameDT=off
  Switch1 : Switch  Criteria=u2 > Threshold  SaturateOnIntegerOverflow=off  InputSameDT=off
  Unit Delay1 : UnitDelay  InitialCondition=LPFvRate2PitchInit*pi/180  SampleTime=-1  HasFrameUpgradeWarning=on
  a1 : Gain  Gain=1-Fp_Elevator
  b0 : Gain  Gain=Fp_Elevator
  Output : Outport  VectorParamsAs1DForOutWhenUnconnected=off
  wires:
  Constant11/1 -> Compare To Constant2/1
  Compare To Constant2/1 -> Switch1/2
  Switch1/1 -> Output/1
  a1/1 -> Add1/1
  Unit Delay1/1 -> a1/1
  b0/1 -> Add1/2
  Add1/1 -> Switch/3, Switch1/1
  Input/1 -> Switch1/3, b0/1
  Switch/1 -> Unit Delay1/1
  Reset/1 -> Switch/2
  ResetValue/1 -> Switch/1

== system Maneuver/Subsystem/Pitch to Elevator/Pitch Moment Caused By Damping ==
  note: An estimation of damping moment produced proportionally to body pitch rate.
  PitchRate_Body : Inport
  TAS : Inport  Port=2
  AverageWingChord : Constant  Value=c
  Constant : Constant  Value=PitchDamping
  Gain : Gain  Gain=2
  Multiply : Product  Inputs=***/
  DAMP : Outport  VectorParamsAs1DForOutWhenUnconnected=off
  wires:
  AverageWingChord/1 -> Multiply/3
  Gain/1 -> Multiply/4
  Multiply/1 -> DAMP/1
  Constant/1 -> Multiply/1
  TAS/1 -> Gain/1
  PitchRate_Body/1 -> Multiply/2

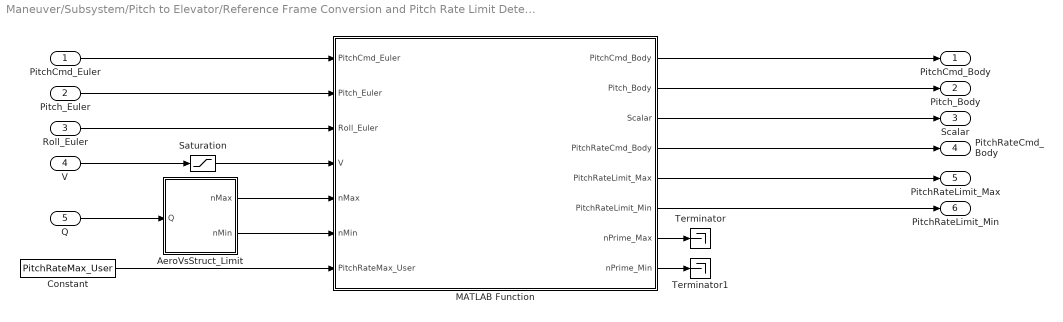
== system Maneuver/Subsystem/Pitch to Elevator/Reference Frame Conversion and Pitch Rate Limit Determination ==
  PitchCmd_Euler : Inport
  Pitch_Euler : Inport  Port=2
  Roll_Euler : Inport  Port=3
  V : Inport  Port=4
  Q : Inport  Port=5
  AeroVsStruct_Limit : Subsystem
  Constant : Constant  Value=PitchRateMax_User
  MATLAB Function : MATLAB Function  TreatAsAtomicUnit=on
  Saturation : Saturate  UpperLimit=100  LowerLimit=5
  Terminator : Terminator
  Terminator1 : Terminator
  PitchCmd_Body : Outport  VectorParamsAs1DForOutWhenUnconnected=off
  "Pitch_Body " : Outport  Port=2  VectorParamsAs1DForOutWhenUnconnected=off
  "Scalar " : Outport  Port=3  VectorParamsAs1DForOutWhenUnconnected=off
  PitchRateCmd_Body : Outport  Port=4  VectorParamsAs1DForOutWhenUnconnected=off
  "PitchRateLimit_Max " : Outport  Port=5  VectorParamsAs1DForOutWhenUnconnected=off
  "PitchRateLimit_Min " : Outport  Port=6  VectorParamsAs1DForOutWhenUnconnected=off
  wires:
  Saturation/1 -> MATLAB Function/4(V)
  V/1 -> Saturation/1
  PitchCmd_Euler/1 -> MATLAB Function/1(PitchCmd_Euler)
  Pitch_Euler/1 -> MATLAB Function/2(Pitch_Euler)
  Roll_Euler/1 -> MATLAB Function/3(Roll_Euler)
  MATLAB Function/1(PitchCmd_Body) -> PitchCmd_Body/1
  MATLAB Function/2(Pitch_Body) -> "Pitch_Body "/1
  MATLAB Function/3(Scalar) -> "Scalar "/1
  MATLAB Function/5(PitchRateLimit_Max) -> "PitchRateLimit_Max "/1
  MATLAB Function/6(PitchRateLimit_Min) -> "PitchRateLimit_Min "/1
  Constant/1 -> MATLAB Function/7(PitchRateMax_User)
  MATLAB Function/4(PitchRateCmd_Body) -> PitchRateCmd_Body/1
  AeroVsStruct_Limit/1(nMax) -> MATLAB Function/5(nMax)
  AeroVsStruct_Limit/2("nMin ") -> MATLAB Function/6(nMin)
  Q/1 -> AeroVsStruct_Limit/1(Q)
  MATLAB Function/7(nPrime_Max) -> Terminator/1
  MATLAB Function/8(nPrime_Min) -> Terminator1/1

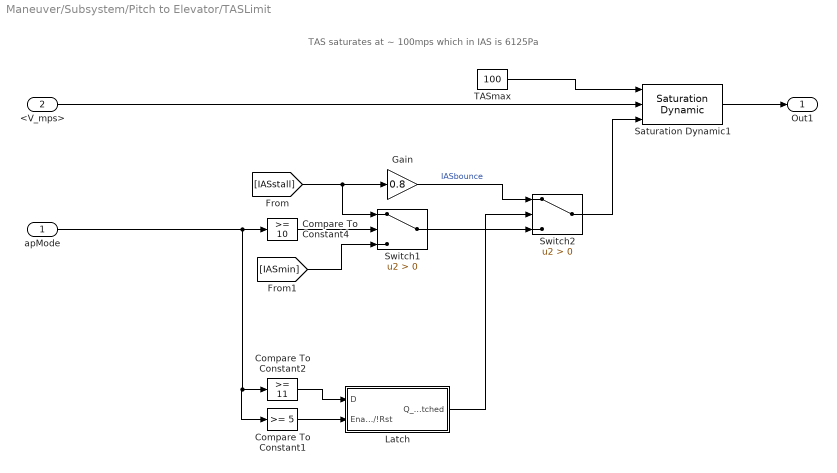
== system Maneuver/Subsystem/Pitch to Elevator/TASLimit ==
  note: TAS saturates at ~ 100mps which in IAS is 6125Pa
  apMode : Inport
  <V_mps> : Inport  Port=2
  Compare To Constant1 : simulink/Logic and Bit Operations/Compare To Constant  relop=>=  const=5  OutDataTypeStr=uint8
  Compare To Constant2 : simulink/Logic and Bit Operations/Compare To Constant  relop=>=  const=11  OutDataTypeStr=uint8
  Compare To Constant4 : simulink/Logic and Bit Operations/Compare To Constant  relop=>=  const=10  OutDataTypeStr=uint8
  Gain : Gain  Gain=0.8
  Latch : Subsystem
  Saturation Dynamic1 : simulink/Discontinuities/Saturation Dynamic  OutMin=[]  OutMax=[]  OutDataTypeStr=Inherit: Same as second input  OutDataType=fixdt(1, 16)  OutScaling=2^-10  DoSatur=off
  Switch1 : Switch  Criteria=u2 > Threshold  SaturateOnIntegerOverflow=off  InputSameDT=off
  Switch2 : Switch  Criteria=u2 > Threshold  SaturateOnIntegerOverflow=off  InputSameDT=off
  TASmax : Constant  Value=100
  Out1 : Outport  VectorParamsAs1DForOutWhenUnconnected=off
  wires:
  Switch2/1 -> Saturation Dynamic1/3
  Compare To Constant4/1 -> Switch1/2
  [IASstall] -> Gain/1, Switch1/1
  Saturation Dynamic1/1 -> Out1/1
  [IASmin] -> Switch1/3
  <V_mps>/1 -> Saturation Dynamic1/2
  Latch/1(Q_Latched) -> Switch2/2
  Compare To Constant2/1 -> Latch/1(D)
  apMode/1 -> Compare To Constant1/1, Compare To Constant2/1, Compare To Constant4/1
  Switch1/1 -> Switch2/3
  Compare To Constant1/1 -> Latch/2(Enable/!Rst)
  Gain/1 -> Switch2/1  "IASbounce"
  TASmax/1 -> Saturation Dynamic1/1

== system Maneuver/Subsystem/Pitch to Elevator/Triggered Subsystem ==
  In1 : Inport
  Trigger : TriggerPort  TriggerType=falling  VariantControl=Variant
  Out1 : Outport  VectorParamsAs1DForOutWhenUnconnected=off
  wires:
  In1/1 -> Out1/1

== system Maneuver/Subsystem/Pitch to Elevator/resetCondition ==
  Compare To Constant1 : simulink/Logic and Bit Operations/Compare To Constant  relop=<=  const=2  OutDataTypeStr=uint8
  Compare To Constant3 : simulink/Logic and Bit Operations/Compare To Constant  relop===  const=11  OutDataTypeStr=uint8
  NOT : Logic  Operator=NOT  IconShape=distinctive  AllPortsSameDT=off  OutDataTypeStr=boolean
  OR : Logic  Operator=OR  Inputs=3  IconShape=distinctive  AllPortsSameDT=off  OutDataTypeStr=boolean
  reset : Outport  VectorParamsAs1DForOutWhenUnconnected=off
  wires:
  [Pic_AP_Mode] -> Compare To Constant1/1, Compare To Constant3/1
  Compare To Constant3/1 -> OR/1
  OR/1 -> reset/1  "Sim.KI_Pitch_Reset"
  Compare To Constant1/1 -> OR/2
  [ApGlobal] -> NOT/1
  NOT/1 -> OR/3

== system Maneuver/Subsystem/Pitch to Elevator/resetVal ==
  note: This init value is intended to aid trimming at start of in-flight simulation and should not be used for reset during liftoffs/bouncing. Will use 0 as alternative reset value as was done previously
  Constant1 : Constant  Value=Pitch2ElevatorIntegratorInit
  Constant2 : Constant  Value=0
  Constant3 : Constant  Value=0
  Switch : Switch  Threshold=9  SaturateOnIntegerOverflow=off  InputSameDT=off
  Switch1 : Switch  Threshold=3  SaturateOnIntegerOverflow=off  InputSameDT=off
  resetVal : Outport  VectorParamsAs1DForOutWhenUnconnected=off
  wires:
  Constant2/1 -> Switch/1
  [Pic_AP_Mode] -> Switch1/2, Switch/2
  Switch/1 -> resetVal/1
  Constant1/1 -> Switch1/1
  Switch1/1 -> Switch/3
  Constant3/1 -> Switch1/3

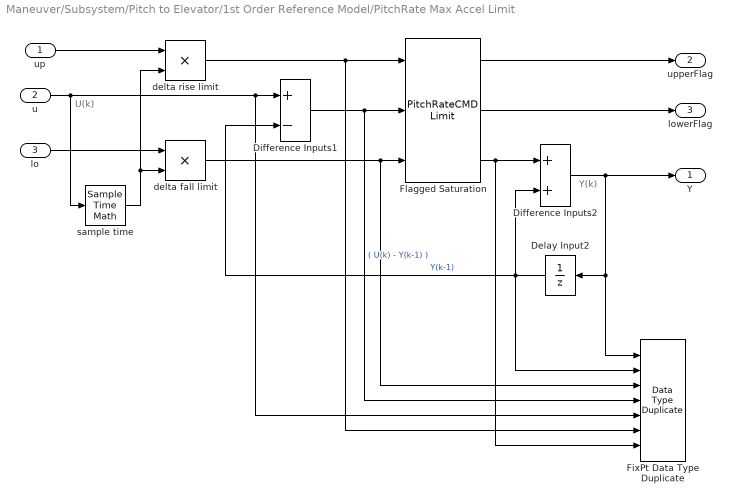
== system Maneuver/Subsystem/Pitch to Elevator/1st Order Reference Model/PitchRate Max Accel Limit ==
  note: Y(k)
  note: U(k)
  up : Inport
  u : Inport  Port=2
  lo : Inport  Port=3
  Delay Input2 : UnitDelay  Description=Store in Global RAM  DisableCoverage=on  InitialCondition=RateLimitPitchRateAccel  SampleTime=-1  HasFrameUpgradeWarning=on
  Difference Inputs1 : Sum  Description=Add in CPU  DisableCoverage=on  Inputs=+-  OutDataTypeStr=Inherit: Inherit via back propagation
  Difference Inputs2 : Sum  Description=Add in CPU  OutDataTypeStr=Inherit: Inherit via back propagation
  FixPt Data Type Duplicate : DataTypeDuplicate  DisableCoverage=on  NumInputPorts=7
  Flagged Saturation : Lib_Piccolo/Pitch to Elevator/1st Order Reference Model/PitchRateCMD Limit  SystemSampleTime=-1  VariantActivationTime=update diagram  AllowFlexibleInterface=on  Latency=0  AutoFrameSizeCalculation=off
  delta fall limit : Product  DisableCoverage=on  Inputs=**  OutDataTypeStr=Inherit: Inherit via back propagation  SaturateOnIntegerOverflow=on
  delta rise limit : Product  DisableCoverage=on  Inputs=**  OutDataTypeStr=Inherit: Inherit via back propagation  SaturateOnIntegerOverflow=on
  sample time : SampleTimeMath  DisableCoverage=on  TsampMathOp=Ts Only  weightValue=1
  Y : Outport  InitialOutput=0  VectorParamsAs1DForOutWhenUnconnected=off
  upperFlag : Outport  Port=2  VectorParamsAs1DForOutWhenUnconnected=off
  lowerFlag : Outport  Port=3  VectorParamsAs1DForOutWhenUnconnected=off
  wires:
  Flagged Saturation/2 -> lowerFlag/1
  Flagged Saturation/1 -> upperFlag/1
  Difference Inputs2/1 -> Y/1, FixPt Data Type Duplicate/1, Delay Input2/1
  sample time/1 -> delta rise limit/2, delta fall limit/2
  Delay Input2/1 -> FixPt Data Type Duplicate/2, Difference Inputs1/2, Difference Inputs2/2  "Y(k-1)"
  up/1 -> delta rise limit/1
  u/1 -> sample time/1, FixPt Data Type Duplicate/5, Difference Inputs1/1
  Flagged Saturation/3 -> Difference Inputs2/1, FixPt Data Type Duplicate/7
  lo/1 -> delta fall limit/1
  delta rise limit/1 -> Flagged Saturation/1, FixPt Data Type Duplicate/6
  Difference Inputs1/1 -> FixPt Data Type Duplicate/4, Flagged Saturation/2  "( U(k) - Y(k-1) )"
  delta fall limit/1 -> FixPt Data Type Duplicate/3, Flagged Saturation/3

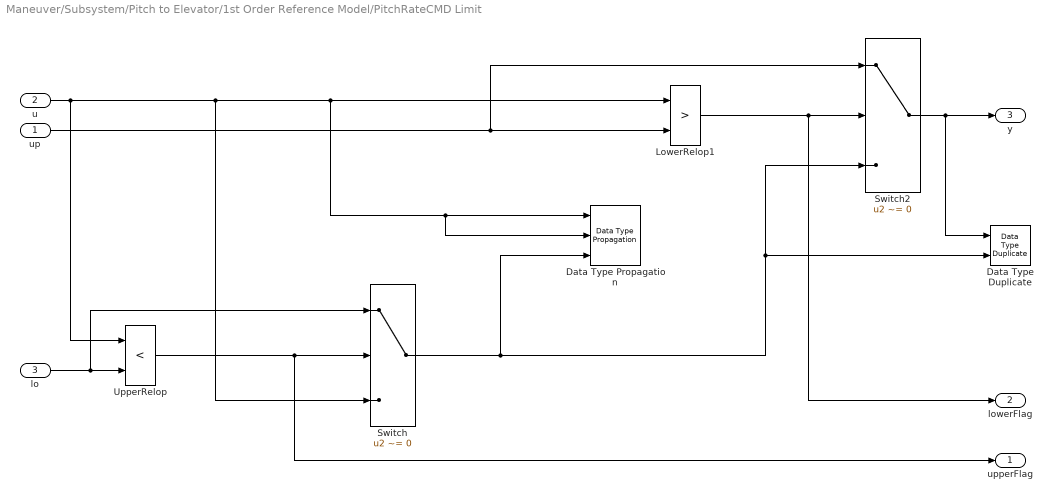
== system Maneuver/Subsystem/Pitch to Elevator/1st Order Reference Model/PitchRateCMD Limit ==
  up : Inport
  u : Inport  Port=2
  lo : Inport  Port=3
  Data Type Duplicate : DataTypeDuplicate  DisableCoverage=on
  Data Type Propagation : simulink/Signal Attributes/Data Type Propagation  PropDataType=fixdt(1, 16)  IfRefDouble=double  IfRefSingle=single  IsSigned=IsSigned1  NumBitsBase=NumBits1  NumBitsMult=1  NumBitsAdd=0  NumBitsAllowFinal=1:128  PropScaling=2^-10  ValuesUsedBestPrec=[5 -7]  SlopeBase=Slope1  SlopeMult=1  SlopeAdd=0  BiasBase=Bias1  BiasMult=1  BiasAdd=0
  LowerRelop1 : RelationalOperator  DisableCoverage=on  Operator=>  OutDataTypeStr=boolean  InputSameDT=off
  Switch : Switch  Criteria=u2 ~= 0  OutDataTypeStr=Inherit: Inherit via back propagation  ZeroCross=off  SaturateOnIntegerOverflow=off  InputSameDT=off
  Switch2 : Switch  Criteria=u2 ~= 0  OutDataTypeStr=Inherit: Inherit via back propagation  ZeroCross=off  SaturateOnIntegerOverflow=off  InputSameDT=off
  UpperRelop : RelationalOperator  DisableCoverage=on  Operator=<  OutDataTypeStr=boolean  InputSameDT=off
  upperFlag : Outport  VectorParamsAs1DForOutWhenUnconnected=off
  lowerFlag : Outport  Port=2  VectorParamsAs1DForOutWhenUnconnected=off
  y : Outport  Port=3  VectorParamsAs1DForOutWhenUnconnected=off
  wires:
  up/1 -> LowerRelop1/2, Switch2/1
  Switch2/1 -> y/1, Data Type Duplicate/1
  u/1 -> UpperRelop/1, Switch/3, LowerRelop1/1, Data Type Propagation/1, Data Type Propagation/2
  lo/1 -> UpperRelop/2, Switch/1
  LowerRelop1/1 -> lowerFlag/1, Switch2/2
  Switch/1 -> Data Type Propagation/3, Switch2/3, Data Type Duplicate/2
  UpperRelop/1 -> upperFlag/1, Switch/2

== system Maneuver/Subsystem/Pitch to Elevator/1st Order Reference Model/resetCondition ==
  apMode : Inport
  Compare To Constant1 : simulink/Logic and Bit Operations/Compare To Constant  relop=<=  const=2  OutDataTypeStr=uint8
  Compare To Constant3 : simulink/Logic and Bit Operations/Compare To Constant  relop===  const=11  OutDataTypeStr=uint8
  NOT : Logic  Operator=NOT  IconShape=distinctive  AllPortsSameDT=off  OutDataTypeStr=boolean
  OR : Logic  Operator=OR  Inputs=3  IconShape=distinctive  AllPortsSameDT=off  OutDataTypeStr=boolean
  Reset : Outport  VectorParamsAs1DForOutWhenUnconnected=off
  wires:
  apMode/1 -> Compare To Constant1/1, Compare To Constant3/1
  Compare To Constant3/1 -> OR/1
  OR/1 -> Reset/1
  Compare To Constant1/1 -> OR/2
  [ApGlobal] -> NOT/1
  NOT/1 -> OR/3

== system Maneuver/Subsystem/Pitch to Elevator/Cm//Alpha Estimation/LPF CLest ==
  Input : Inport
  Reset : Inport  Port=2
  Add1 : Sum  Inputs=++|
  Compare To Constant2 : simulink/Logic and Bit Operations/Compare To Constant  relop=>  const=0  OutDataTypeStr=uint8
  Constant11 : Constant  Value=PB/gain_resolution(4)
  "LPF " : DiscreteTransferFcn  Commented=on  Numerator=[(2*Fp_Pitch_2) 0]  Denominator=[1 (2*Fp_Pitch_2-1)]  InitialStates=3
  Switch1 : Switch  Criteria=u2 > Threshold  SaturateOnIntegerOverflow=off  InputSameDT=off
  Unit Delay1 : UnitDelay  InitialCondition=LPFclestInit  SampleTime=-1  HasFrameUpgradeWarning=on
  a1 : Gain  Gain=1-(2*(0.55*2*pi*PB/gain_resolution(4)*dt))
  b0 : Gain  Gain=(2*(0.55*2*pi*PB/gain_resolution(4)*dt))
  Output : Outport  VectorParamsAs1DForOutWhenUnconnected=off
  wires:
  Constant11/1 -> Compare To Constant2/1
  Compare To Constant2/1 -> Switch1/2
  Switch1/1 -> Output/1
  Input/1 -> b0/1, Switch1/3
  Add1/1 -> Switch1/1, Unit Delay1/1
  a1/1 -> Add1/1
  b0/1 -> Add1/2
  Unit Delay1/1 -> a1/1

== system Maneuver/Subsystem/Pitch to Elevator/DynamicPLimit/Latch ==
  D : Inport
  Enable/!Rst : Inport  Port=2
  AND : Logic  IconShape=distinctive  AllPortsSameDT=off  OutDataTypeStr=boolean
  Constant : Constant
  OR : Logic  Operator=OR  IconShape=distinctive  AllPortsSameDT=off  OutDataTypeStr=boolean
  Switch : Switch  Criteria=u2 > Threshold  Threshold=0.5  SaturateOnIntegerOverflow=off  InputSameDT=off
  Unit Delay : UnitDelay  SampleTime=-1  HasFrameUpgradeWarning=on
  Q_Latched : Outport  VectorParamsAs1DForOutWhenUnconnected=off
  wires:
  Unit Delay/1 -> OR/2
  Switch/1 -> Q_Latched/1, Unit Delay/1
  D/1 -> Switch/3, OR/1
  OR/1 -> AND/1
  AND/1 -> Switch/2
  Enable/!Rst/1 -> AND/2
  Constant/1 -> Switch/1

== system Maneuver/Subsystem/Pitch to Elevator/Elevator Ramp Logic/Elevator DeRotation Ramp ==
  Elevator In : Inport
  apMode In : Inport  Port=2
  Compare To Constant2 : simulink/Logic and Bit Operations/Compare To Constant  relop===  const=11  OutDataTypeStr=uint8
  Constant : Constant  Value=ElevatorDeflectionRate
  Discrete-Time Integrator : DiscreteIntegrator  ExternalReset=rising  InitialConditionSource=external  SampleTime=-1  LimitOutput=on  UpperSaturationLimit=RollingElevator  LowerSaturationLimit=-ElevatorMax  ICPrevOutput=DiscIntNeverNeededParam  ICPrevScaledInput=DiscIntNeverNeededParam
  NOT : Logic  Operator=NOT  IconShape=distinctive  AllPortsSameDT=off  OutDataTypeStr=boolean
  Switch : Switch  Criteria=u2 > Threshold  SaturateOnIntegerOverflow=off  InputSameDT=off
  Unit Delay : UnitDelay  SampleTime=-1  HasFrameUpgradeWarning=on
  Elevator Out : Outport  VectorParamsAs1DForOutWhenUnconnected=off
  wires:
  Discrete-Time Integrator/1 -> Switch/3  "Sim.rampElevator"
  Constant/1 -> Discrete-Time Integrator/1
  Elevator In/1 -> Unit Delay/1, Switch/1
  NOT/1 -> Switch/2
  Switch/1 -> Elevator Out/1
  Unit Delay/1 -> Discrete-Time Integrator/3
  apMode In/1 -> Compare To Constant2/1
  Compare To Constant2/1 -> Discrete-Time Integrator/2, NOT/1

== system Maneuver/Subsystem/Pitch to Elevator/Elevator Ramp Logic/Elevator Rotation Ramp ==
  Elevator In : Inport
  apMode In : Inport  Port=2
  Compare To Constant2 : simulink/Logic and Bit Operations/Compare To Constant  relop===  const=2  OutDataTypeStr=uint8
  Constant : Constant  Value=RotationRate
  Constant1 : Constant  Value=LaunchRollingElevator
  Constant2 : Constant  Value=LaunchRollingElevator
  Discrete-Time Integrator : DiscreteIntegrator  ExternalReset=rising  InitialConditionSource=external  SampleTime=-1  LimitOutput=on  UpperSaturationLimit=LaunchRollingElevator  LowerSaturationLimit=RotationElevator  ICPrevOutput=DiscIntNeverNeededParam  ICPrevScaledInput=DiscIntNeverNeededParam
  NOT : Logic  Operator=NOT  IconShape=distinctive  AllPortsSameDT=off  OutDataTypeStr=boolean
  Switch : Switch  Criteria=u2 > Threshold  SaturateOnIntegerOverflow=off  InputSameDT=off
  Switch1 : Switch  Threshold=2  SaturateOnIntegerOverflow=off  InputSameDT=off
  Elevator Out : Outport  VectorParamsAs1DForOutWhenUnconnected=off
  wires:
  Discrete-Time Integrator/1 -> Switch/3  "Sim.RotationRampElevator"
  Constant/1 -> Discrete-Time Integrator/1
  Elevator In/1 -> Switch/1
  NOT/1 -> Switch/2
  Constant2/1 -> Discrete-Time Integrator/3
  apMode In/1 -> Switch1/2, Compare To Constant2/1
  Compare To Constant2/1 -> Discrete-Time Integrator/2, NOT/1
  Switch/1 -> Switch1/1
  Switch1/1 -> Elevator Out/1
  Constant1/1 -> Switch1/3
